simulink model "BLDC_model_My_model"  (R2024b)
settings: Solver=VariableStepAuto  StartTime=0.0  StopTime=2  FixedStep=1e-5  MaxStep=1e-5  RelTol=1e-3
model workspace (MAT data in the model file):
  B = 1e-06
  J = 5e-06
  Ke = 0.0006
  Ls = 2e-05
  Pm = 0.0006
  Rs = 0.06
  f = 50
  p = 8
libraries: spsMosfetLib x6, spsVoltageMeasurementLib x3, dspstat3 x1, slpidlib x1, spsControlledVoltageSourceLib x1, spsDCVoltageSourceLib x1, ee_lib x1, spspowerguiLib x1
settings Model: Creator=ahmed  LastModifiedBy=ahmed

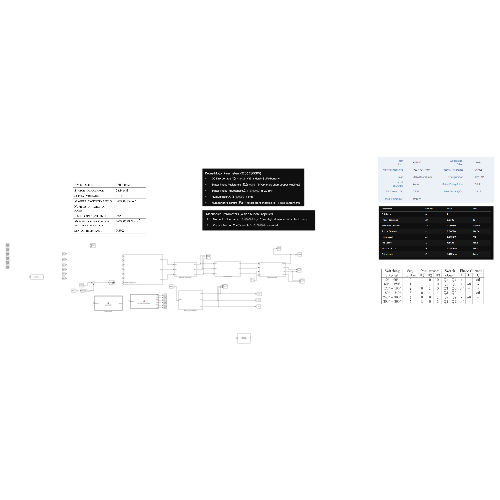
[thumbnail: Simulink's stored preview of the top-level diagram]
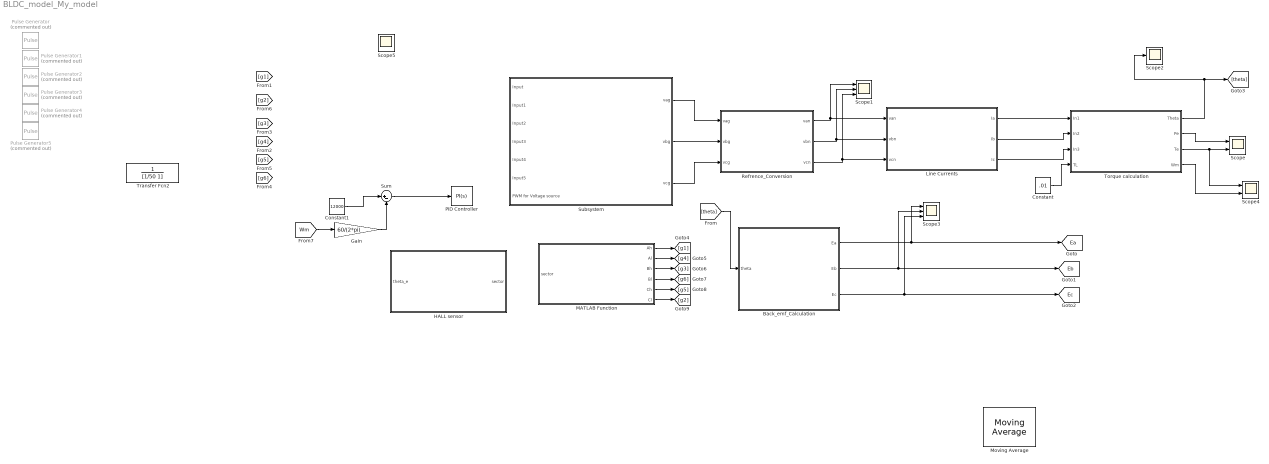
== system BLDC_model_My_model ==
  Back_emf_Calculation : Subsystem
  Constant : Constant  Value=.01
  Constant1 : Constant  Value=12000
  Gain : Gain  Gain=60/(2*pi)
  HALL sensor : MATLAB Function  TreatAsAtomicUnit=on
  Line Currents : Subsystem
  MATLAB Function : MATLAB Function  TreatAsAtomicUnit=on
  Moving Average : dspstat3/Moving Average  Method=Sliding window  ForgettingFactorPort=off  SpecifyWindowLength=on  WindowLength=4  OverlapLength=3  AllowArbitraryInputLength=off  ForgettingFactor=0.9  SimulateUsing=Interpreted execution
  PID Controller : slpidlib/PID Controller  Controller=PI  Form=Parallel  TimeDomain=Continuous-time  UseExternalTs=off  SampleTime=-1  IntegratorMethod=Forward Euler  FilterMethod=Forward Euler  ControllerParametersSource=internal  P=.02  I=600  UseKiTs=off  D=0  UseExternalDerivativeSource=off  N=100  UseFilter=on  TunerSelectOption=Transfer Function Based (PID Tuner App)  InitialConditionSource=internal  InitialConditionForIntegrator=0  InitialConditionForFilter=0  DifferentiatorICPrevScaledInput=0  ExternalReset=none  TrackingMode=off  Kt=1  LimitOutput=on  SatLimitsSource=internal  UpperSaturationLimit=0.636 * 24  LowerSaturationLimit=0  LinearizeAsGain=on  AntiWindupMode=clamping  Kb=1  LimitIntegrator=off  UpperIntegratorSaturationLimit=inf  LowerIntegratorSaturationLimit=-inf  POutMin=[]  POutMax=[]  IOutMin=[]  IOutMax=[]  DOutMin=[]  DOutMax=[]  NOutMin=[]  NOutMax=[]  SumOutMin=[]  SumOutMax=[]  SaturationOutMin=[]  SaturationOutMax=[]  PParamMin=[]  PParamMax=[]  IParamMin=[]  IParamMax=[]  DParamMin=[]  DParamMax=[]  NParamMin=[]  NParamMax=[]  KbParamMin=[]  KbParamMax=[]  KtParamMin=[]  KtParamMax=[]  KbOutMin=[]  KbOutMax=[]  KtOutMin=[]  KtOutMax=[]  IntegratorOutMin=[]  IntegratorOutMax=[]  FilterOutMin=[]  FilterOutMax=[]  SumI1OutMin=[]  SumI1OutMax=[]  SumI2OutMin=[]  SumI2OutMax=[]  SumI3OutMin=[]  SumI3OutMax=[]  SumI4OutMin=[]  SumI4OutMax=[]  SumDOutMin=[]  SumDOutMax=[]  DifferentiatorOutMin=[]  DifferentiatorOutMax=[]  FilterDiffOutCoefMin=[]  FilterDiffOutCoefMax=[]  ReciprocalOutMin=[]  ReciprocalOutMax=[]  SumDenOutMin=[]  SumDenOutMax=[]  SumNumOutMin=[]  SumNumOutMax=[]  DivideOutMin=[]  DivideOutMax=[]  UdiffTsProdOutMin=[]  UdiffTsProdOutMax=[]  NTsProdOutMin=[]  NTsProdOutMax=[]  UintegralTsProdOutMin=[]  UintegralTsProdOutMax=[]  UngainTsProdOutMin=[]  UngainTsProdOutMax=[]  ClampingZeroOutDataTypeStr=Inherit: Inherit via back propagation  ClampingZeroOutMin=[]  ClampingZeroOutMax=[]  FilterDenConstantOutDataTypeStr=Inherit: Inherit via back propagation  FilterDenConstantOutMin=[]  FilterDenConstantOutMax=[]  PCopyOutDataTypeStr=Inherit: Inherit via back propagation  PCopyOutMin=[]  PCopyOutMax=[]  NCopyOutDataTypeStr=Inherit: Inherit via back propagation  NCopyOutMin=[]  NCopyOutMax=[]  IntegratorContinuousStateAttributes=''  IntegratorStateMustResolveToSignalObject=off  IntegratorRTWStateStorageClass=Auto  FilterContinuousStateAttributes=''  FilterStateMustResolveToSignalObject=off  FilterRTWStateStorageClass=Auto  ParallelPVariant=InternalParameters  IdealPVariant=Disabled  IVariant=InternalParameters  DVariant=Disabled  IntegratorVariant=Continuous  SatVariant=Enabled  AWVariant=ContClampingParallel  PCopyVariant=Disabled  TRVariant=Disabled  FdbkBlocksVariant=Forward  IdealPFdbkVariant=Disabled  SatFdbkVariant=Disabled  DerivativeFilterVariant=Disabled  NVariant=Disabled  NCopyVariant=Disabled_SignalSpec  FilterICVariant=Disabled  IntegratorICVariant=InternalICs  ExternalResetVariant=Disabled  TRSumVariant=Passthrough  SumFdbkVariant=Disabled  SumVariant=Sum_PI  TsampFilterVariant=InternalTs  TsampNgainVariant=Passthrough  TsampIntegralVariant=Disabled_SignalSpec  ExternalSaturationOutDataTypeStr=Inherit: Same as second input  DerivativeSourceVariant=Disabled  PreIntVariant=InternalPreInt
  Pulse Generator : DiscretePulseGenerator  Commented=on  PulseType=Time based  Period=1/f  PulseWidth=33
  Pulse Generator1 : DiscretePulseGenerator  Commented=on  PulseType=Time based  Period=1/f  PulseWidth=33  PhaseDelay=2*(1/f)/3
  Pulse Generator2 : DiscretePulseGenerator  Commented=on  PulseType=Time based  Period=1/f  PulseWidth=33  PhaseDelay=(1/f)/3
  Pulse Generator3 : DiscretePulseGenerator  Commented=on  PulseType=Time based  Period=1/f  PulseWidth=33  PhaseDelay=(1/f)/2
  Pulse Generator4 : DiscretePulseGenerator  Commented=on  PulseType=Time based  Period=1/f  PulseWidth=33  PhaseDelay=(1/f)/6
  Pulse Generator5 : DiscretePulseGenerator  Commented=on  PulseType=Time based  Period=1/f  PulseWidth=33  PhaseDelay=5*(1/f)/6
  Refrence_Conversion : Subsystem
  Scope : Scope  NumInputPorts=2
  Scope1 : Scope  NumInputPorts=3
  Scope2 : Scope
  Scope3 : Scope  NumInputPorts=3
  Scope4 : Scope  NumInputPorts=2
  Scope5 : Scope  NumInputPorts=3
  Subsystem : Subsystem
  Sum : Sum  Inputs=|+-
  Torque calculation : Subsystem
  Transfer Fcn2 : TransferFcn  Denominator=[1/50 1]
  tag scope: Ea=global, Eb=global, Ec=global
  wires:
  Subsystem/2(vbg) -> Refrence_Conversion/2(vbg)
  Subsystem/1(vag) -> Refrence_Conversion/1(vag)
  Subsystem/3(vcg) -> Refrence_Conversion/3(vcg)
  Refrence_Conversion/1(van) -> Scope1/1, Line Currents/1(van)
  Refrence_Conversion/2(vbn) -> Scope1/2, Line Currents/2(vbn)
  Refrence_Conversion/3(vcn) -> Scope1/3, Line Currents/3(vcn)
  Line Currents/1(Ia) -> Torque calculation/1(In1)
  Line Currents/2(Ib) -> Torque calculation/2(In2)
  Line Currents/3(Ic) -> Torque calculation/3(In3)
  Torque calculation/1(Theta) -> Scope2/1, [theta]
  Back_emf_Calculation/1(Ea) -> [Ea], Scope3/1
  Back_emf_Calculation/3(Ec) -> [Ec], Scope3/3
  Back_emf_Calculation/2(Eb) -> [Eb], Scope3/2
  MATLAB Function/1(Ah) -> [g1]
  MATLAB Function/2(Al) -> [g4]
  MATLAB Function/3(Bh) -> [g3]
  MATLAB Function/4(Bl) -> [g6]
  MATLAB Function/5(Ch) -> [g5]
  MATLAB Function/6(Cl) -> [g2]
  Torque calculation/2(Pe) -> Scope/1
  Torque calculation/3(Te) -> Scope4/1, Scope/2
  Torque calculation/4(Wm) -> Scope4/2
  Constant/1 -> Torque calculation/4(TL)
  Sum/1 -> PID Controller/1
  [Wm] -> Gain/1
  Gain/1 -> Sum/2
  Constant1/1 -> Sum/1
  [theta] -> Back_emf_Calculation/1(theta)

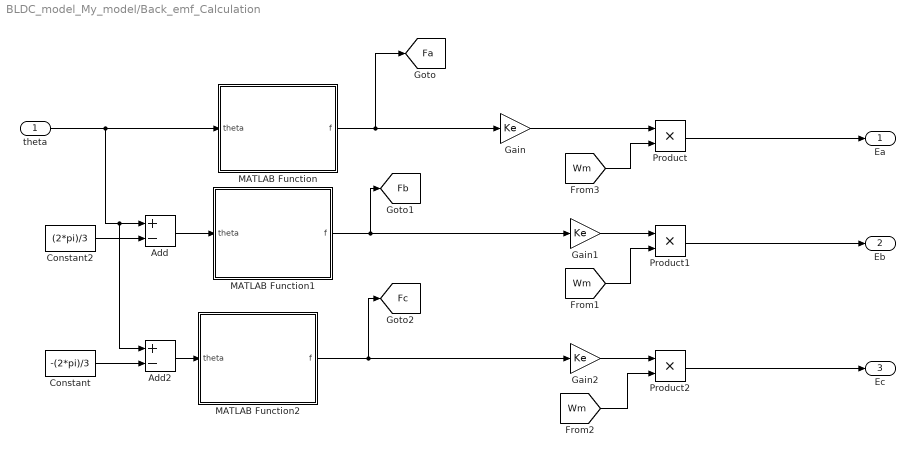
== system BLDC_model_My_model/Back_emf_Calculation ==
  theta : Inport
  Add : Sum  Inputs=+-
  Add2 : Sum  Inputs=+-
  Constant : Constant  Value=-(2*pi)/3
  Constant2 : Constant  Value=(2*pi)/3
  Gain : Gain  Gain=Ke
  Gain1 : Gain  Gain=Ke
  Gain2 : Gain  Gain=Ke
  MATLAB Function : MATLAB Function  TreatAsAtomicUnit=on
  MATLAB Function1 : MATLAB Function  TreatAsAtomicUnit=on
  MATLAB Function2 : MATLAB Function  TreatAsAtomicUnit=on
  Product : Product
  Product1 : Product
  Product2 : Product
  Ea : Outport
  Eb : Outport  Port=2
  Ec : Outport  Port=3
  tag scope: Fa=global, Fb=global, Fc=global
  wires:
  theta/1 -> Add2/1, Add/1, MATLAB Function/1(theta)
  Constant/1 -> Add2/2
  Constant2/1 -> Add/2
  Add/1 -> MATLAB Function1/1(theta)
  Add2/1 -> MATLAB Function2/1(theta)
  MATLAB Function/1(f) -> [Fa], Gain/1
  MATLAB Function1/1(f) -> [Fb], Gain1/1
  MATLAB Function2/1(f) -> [Fc], Gain2/1
  [Wm] -> Product/2
  Gain/1 -> Product/1
  Gain1/1 -> Product1/1
  [Wm] -> Product1/2
  Gain2/1 -> Product2/1
  [Wm] -> Product2/2
  Product/1 -> Ea/1
  Product1/1 -> Eb/1
  Product2/1 -> Ec/1

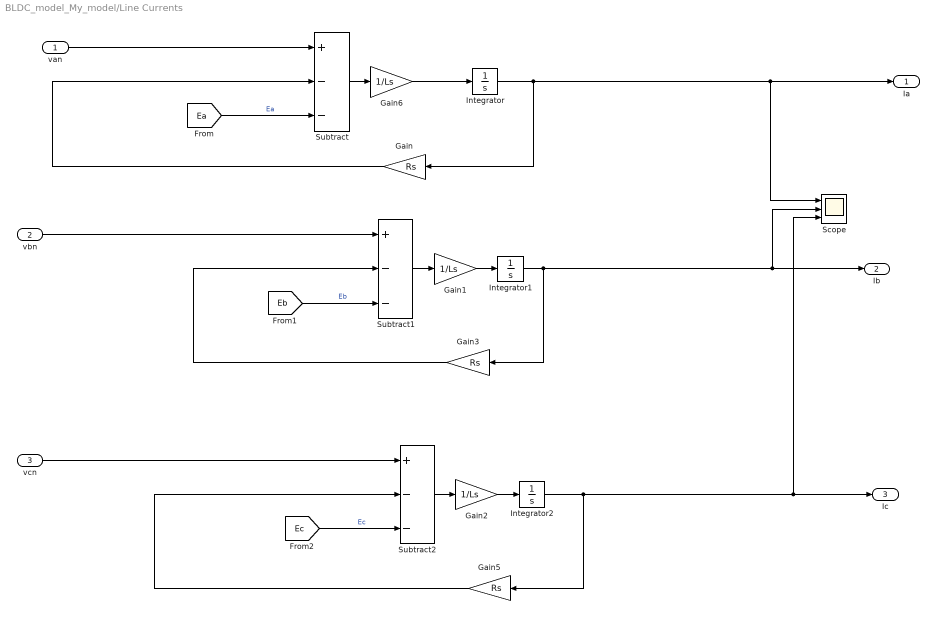
== system BLDC_model_My_model/Line Currents ==
  van : Inport
  vbn : Inport  Port=2
  vcn : Inport  Port=3
  Gain : Gain  Gain=Rs
  Gain1 : Gain  Gain=1/Ls
  Gain2 : Gain  Gain=1/Ls
  Gain3 : Gain  Gain=Rs
  Gain5 : Gain  Gain=Rs
  Gain6 : Gain  Gain=1/Ls
  Integrator : Integrator
  Integrator1 : Integrator
  Integrator2 : Integrator
  Scope : Scope  NumInputPorts=3
  Subtract : Sum  Inputs=+--
  Subtract1 : Sum  Inputs=+--
  Subtract2 : Sum  Inputs=+--
  Ia : Outport
  Ib : Outport  Port=2
  Ic : Outport  Port=3
  wires:
  van/1 -> Subtract/1
  [Ea] -> Subtract/3  "Ea"
  Subtract/1 -> Gain6/1
  Gain/1 -> Subtract/2
  Integrator/1 -> Scope/1, Ia/1, Gain/1
  Gain3/1 -> Subtract1/2
  Subtract1/1 -> Gain1/1
  vbn/1 -> Subtract1/1
  vcn/1 -> Subtract2/1
  Subtract2/1 -> Gain2/1
  Gain5/1 -> Subtract2/2
  [Eb] -> Subtract1/3  "Eb"
  [Ec] -> Subtract2/3  "Ec"
  Integrator2/1 -> Ic/1, Scope/3, Gain5/1
  Integrator1/1 -> Scope/2, Ib/1, Gain3/1
  Gain6/1 -> Integrator/1
  Gain1/1 -> Integrator1/1
  Gain2/1 -> Integrator2/1

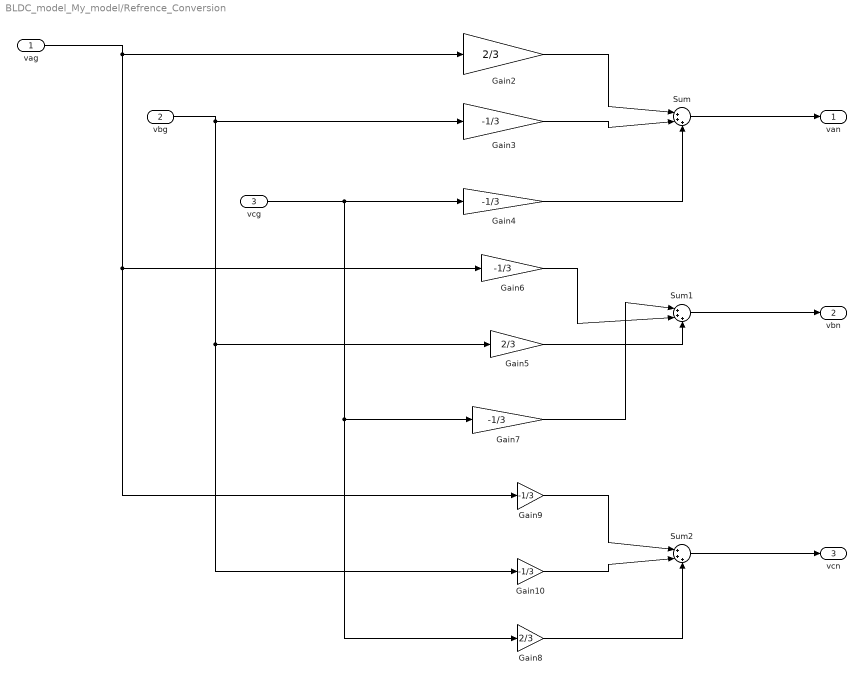
== system BLDC_model_My_model/Refrence_Conversion ==
  vag : Inport
  vbg : Inport  Port=2
  vcg : Inport  Port=3
  Gain{3..4,6..7,9..10} (6 alike) : Gain  Gain=-1/3
  Gain2 : Gain  Gain=2/3
  Gain5 : Gain  Gain=2/3
  Gain8 : Gain  Gain=2/3
  Sum : Sum  Inputs=|+++
  Sum1 : Sum  Inputs=|+++
  Sum2 : Sum  Inputs=|+++
  van : Outport
  vbn : Outport  Port=2
  vcn : Outport  Port=3
  wires:
  Gain10/1 -> Sum2/2
  Gain9/1 -> Sum2/1
  Gain8/1 -> Sum2/3
  Gain7/1 -> Sum1/1
  Gain4/1 -> Sum/3
  Gain3/1 -> Sum/2
  vbg/1 -> Gain10/1, Gain5/1, Gain3/1
  Gain6/1 -> Sum1/2
  Gain2/1 -> Sum/1
  vcg/1 -> Gain8/1, Gain7/1, Gain4/1
  Gain5/1 -> Sum1/3
  vag/1 -> Gain2/1, Gain6/1, Gain9/1
  Sum/1 -> van/1
  Sum1/1 -> vbn/1
  Sum2/1 -> vcn/1

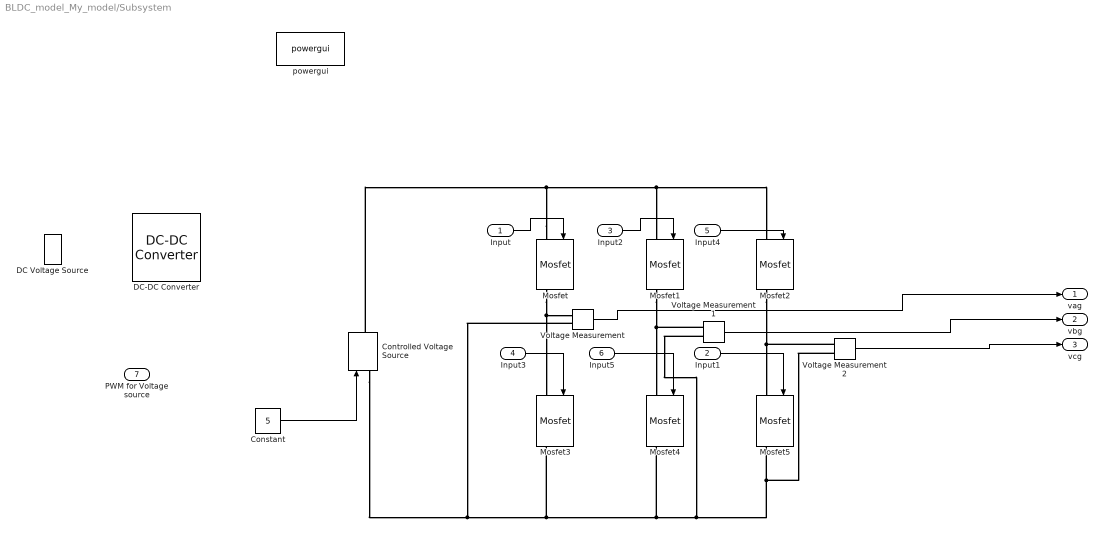
== system BLDC_model_My_model/Subsystem ==
  Input : Inport
  Input1 : Inport  Port=2
  Input2 : Inport  Port=3
  Input3 : Inport  Port=4
  Input4 : Inport  Port=5
  Input5 : Inport  Port=6
  PWM for Voltage source : Inport  Port=7
  Constant : Constant  Value=5
  Controlled Voltage Source : spsControlledVoltageSourceLib/Controlled Voltage Source  Initialize=on  Source_Type=DC  Amplitude=0  Phase=0  Frequency=0  Measurements=Voltage
  DC Voltage Source : spsDCVoltageSourceLib/DC Voltage Source  Amplitude=100  Measurements=None
  DC-DC Converter : ee_lib/Semiconductors & Converters/Converters/DC-DC Converter  Vref_option=ee.enum.converters.voltageref.internal  v_ref=10 V  P_rated=10 W  droop_enabled=true  droop_param=ee.enum.converters.droop.value  droop=0.1 V/A  droop_percent=2  Vref_droop=10 V  reversible=ee.enum.converters.directionality.unidirectional  G_diode=1e-8 1/Ohm  P_fixed=1 W  losses_option=ee.enum.converters.lossesOption.proportionalToSquaredCurrent  eff_rated=80  tableOption=ee.enum.converters.lossTableOptionThermal.currentTemp  i_eff_vec=[-2, -1, 1, 2] A  v_eff_vec=[15, 30, 45] V  eff_vec=[66, 76, 80, 74]  eff_2D_table=[66, 66, 66; 76, 76, 76; 80, 80, 80; 74, 74, 74]  model_dynamics=ee.enum.converters.dynamics.no  tau=0.02 s  v_ini=10 V  v1_min=1 V  R1=1000 Ohm  R2=1000 Ohm  fault_condition=ee.enum.faults.faultInputCondition.greaterThan  fault_threshold=0.5  T_eff_vec=[280, 300, 320] K  eff_3D_table=repmat([66; 76; 80; 74], 1, 3, 3)  thermal_mass=100 J/K  initial_temperature=298.15 K
      settings: InternalSimscapePortConfiguration="{\"Bottom\":[],\"Left\":[{\"id\":\"p1\",\"label\":\"1+\",\"type\":\"foundation.electrical.electrical\"},{\"id\":\"n1\",\"label\":\"1-\",\"type\":\"foundation.electrical.electrical\"}],\"Right\":[{\"id\":\"p2\",\"label\":\"2+\",\"type\":\"foundation.electrical.electrical\"},{\"id\":\"n2\",\"label\":\"2-\",\"type\":\"foundation.electrical.electrical\"}],\"Top\":[]}"
  Mosfet{,1..5} (6 alike) : spsMosfetLib/Mosfet  Ron=0.1  Lon=0  Rd=0.01  Vfd=0  IC=0  Rs=1e5  Cs=inf  Measurements=on
  Voltage Measurement : spsVoltageMeasurementLib/Voltage Measurement  PhasorSimulation=off  OutputType=Complex  PSBequivalent=0
  Voltage Measurement1 : spsVoltageMeasurementLib/Voltage Measurement  PhasorSimulation=off  OutputType=Complex  PSBequivalent=0
  Voltage Measurement2 : spsVoltageMeasurementLib/Voltage Measurement  PhasorSimulation=off  OutputType=Complex  PSBequivalent=0
  powergui : spspowerguiLib/powergui  Priority=1  SimulationMode=Continuous  SampleTime=50e-6  frequency=60  Iterations=50  frequencyindice=0  Pbase=100e6  ErrMax=1e-4  UnitsV=kV  UnitsW=MW  buscounter=0  FunctionMessages=off  echomessages=off  EnableUseOfTLC=off  CurrentSourceSwitches=off  DisableSnubberDevices=off  DisableRonSwitches=off  DisableVfSwitches=off  DisplayEquations=off  AutomaticDiscreteSolvers=off  SolverType=Tustin/Backward Euler (TBE)  Interpol=off  ExternalGateDelay=off  methode=off  Ts=100  x0status=blocks  SPID=on  SwTol=0  HookPort=off  NonlinearTolerance=1e-4  nMaxIteration=100  ContinueOnMaxIteration=off  RestoreLinks=warning  ResistiveCurrentMeasurement=off  Frange=[0:2:500]  Ylog=off  Xlog=on  ShowGrid=off  save=off  variable=ZData  structure=0  ZoomFFT=off  StartTime=0.0  cycles=1  DisplayStyle=1  fundamental=60  FreqAxis=off  MaxFrequency=1000  frequencyindicesteady=1  RmsSteady=1  display=off
  vag : Outport
  vbg : Outport  Port=2
  vcg : Outport  Port=3
  wires:
  Input2/1 -> Mosfet1/1
  Input5/1 -> Mosfet4/1
  Voltage Measurement1/1 -> vbg/1
  Input4/1 -> Mosfet2/1
  Input/1 -> Mosfet/1
  Voltage Measurement/1 -> vag/1
  Input3/1 -> Mosfet3/1
  Input1/1 -> Mosfet5/1
  Voltage Measurement2/1 -> vcg/1
  Constant/1 -> Controlled Voltage Source/1
  connections:
  Mosfet/LConn1 -- Controlled Voltage Source/RConn1 -- Mosfet1/LConn1 -- Mosfet2/LConn1
  Controlled Voltage Source/LConn1 -- Voltage Measurement/LConn2 -- Mosfet3/RConn1 -- Voltage Measurement1/LConn2 -- Voltage Measurement2/LConn2 -- Mosfet5/RConn1 -- Mosfet4/RConn1
  Mosfet2/RConn1 -- Voltage Measurement2/LConn1 -- Mosfet5/LConn1
  Mosfet1/RConn1 -- Voltage Measurement1/LConn1 -- Mosfet4/LConn1
  Mosfet/RConn1 -- Mosfet3/LConn1 -- Voltage Measurement/LConn1

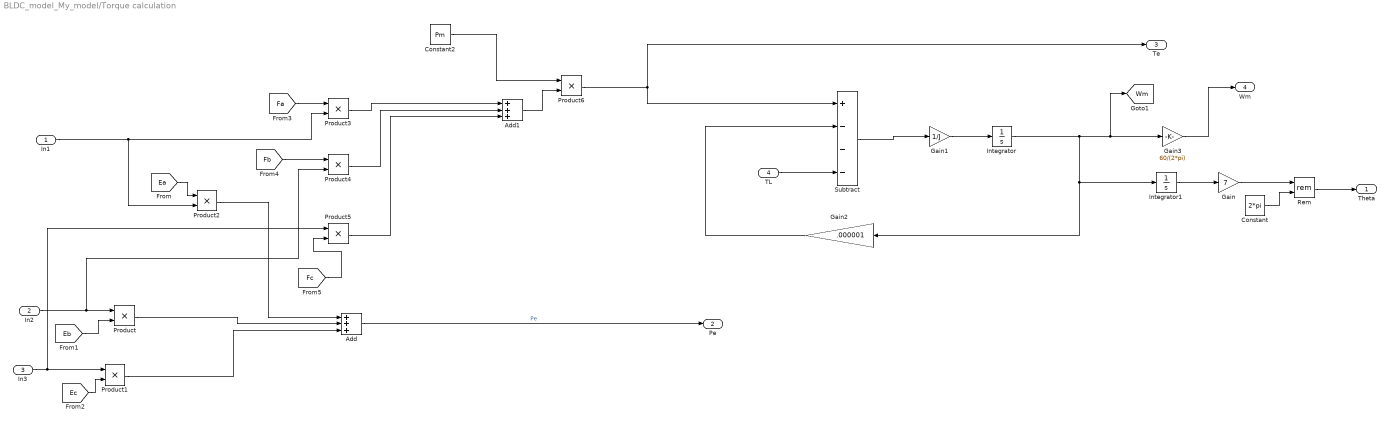
== system BLDC_model_My_model/Torque calculation ==
  In1 : Inport
  In2 : Inport  Port=2
  In3 : Inport  Port=3
  TL : Inport  Port=4
  Add : Sum  Inputs=+++
  Add1 : Sum  Inputs=+++
  Constant : Constant  Value=2*pi
  Constant2 : Constant  Value=Pm
  Gain : Gain  Gain=7
  Gain1 : Gain  Gain=1/J
  Gain2 : Gain  Gain=.000001
  Gain3 : Gain  Gain=60/(2*pi)
  Integrator : Integrator
  Integrator1 : Integrator
  Product{,1..6} (7 alike) : Product
  Rem : Math  Operator=rem
  Subtract : Sum  Inputs=+---
  Theta : Outport
  Pe : Outport  Port=2
  Te : Outport  Port=3
  Wm : Outport  Port=4
  tag scope: Wm=global
  wires:
  In2/1 -> Product4/2, Product/1
  [Eb] -> Product/2
  In3/1 -> Product1/1, Product5/1
  [Ec] -> Product1/2
  [Ea] -> Product2/1
  In1/1 -> Product2/2, Product3/2
  Product2/1 -> Add/1
  Product/1 -> Add/2
  Product1/1 -> Add/3
  Add/1 -> Pe/1  "Pe"
  Integrator1/1 -> Gain/1
  Gain/1 -> Rem/1
  Constant/1 -> Rem/2
  Rem/1 -> Theta/1
  Subtract/1 -> Gain1/1
  Gain1/1 -> Integrator/1
  Integrator/1 -> [Wm], Gain3/1, Integrator1/1, Gain2/1
  Gain2/1 -> Subtract/2
  TL/1 -> Subtract/4
  [Fa] -> Product3/1
  [Fb] -> Product4/1
  [Fc] -> Product5/2
  Product3/1 -> Add1/1
  Product4/1 -> Add1/2
  Product5/1 -> Add1/3
  Add1/1 -> Product6/2
  Constant2/1 -> Product6/1
  Product6/1 -> Te/1, Subtract/1
  Gain3/1 -> Wm/1

== matlab function BLDC_model_My_model/Back_emf_Calculation/MATLAB Function1 ==
  data: theta input; f output
function f = calc_f_standard(theta)
    % calc_f_standard calculates the unit trapezoidal back-EMF waveform 
    % based on the standard literature formulation (starts at the flat top).
    %
    % Input: theta - Electrical angle in radians (can be scalar or array)
    % Output: f - Normalized back-EMF amplitude (-1.0 to 1.0)
    
    % Normalize angle to strictly fall within [0, 2*pi)
    theta_norm = mod(theta, 2*pi);
    
    % Initialize the output array with zeros
    f = zeros(size(theta_norm));
    
    % Region 1: Flat Top (0 to 120 degrees)
    idx = (theta_norm >= 0) & (theta_norm < 2*pi/3);
    f(idx) = 1;
    
    % Region 2: Falling Edge (120 to 180 degrees)
    idx = (theta_norm >= 2*pi/3) & (theta_norm < pi);
    f(idx) = 1 - (6/pi) .* (theta_norm(idx) - 2*pi/3);
    
    % Region 3: Flat Bottom (180 to 300 degrees)
    idx = (theta_norm >= pi) & (theta_norm < 5*pi/3);
    f(idx) = -1;
    
    % Region 4: Rising Edge (300 to 360 degrees)
    idx = (theta_norm >= 5*pi/3) & (theta_norm <= 2*pi);
    f(idx) = -1 + (6/pi) .* (theta_norm(idx) - 5*pi/3);
end

== matlab function BLDC_model_My_model/Back_emf_Calculation/MATLAB Function ==
  data: theta input; f output
function f = calc_f_standard(theta)
    % calc_f_standard calculates the unit trapezoidal back-EMF waveform 
    % based on the standard literature formulation (starts at the flat top).
    %
    % Input: theta - Electrical angle in radians (can be scalar or array)
    % Output: f - Normalized back-EMF amplitude (-1.0 to 1.0)
    
    % Normalize angle to strictly fall within [0, 2*pi)
    theta_norm = mod(theta, 2*pi);
    
    % Initialize the output array with zeros
    f = zeros(size(theta_norm));
    
    % Region 1: Flat Top (0 to 120 degrees)
    idx = (theta_norm >= 0) & (theta_norm < 2*pi/3);
    f(idx) = 1;
    
    % Region 2: Falling Edge (120 to 180 degrees)
    idx = (theta_norm >= 2*pi/3) & (theta_norm < pi);
    f(idx) = 1 - (6/pi) .* (theta_norm(idx) - 2*pi/3);
    
    % Region 3: Flat Bottom (180 to 300 degrees)
    idx = (theta_norm >= pi) & (theta_norm < 5*pi/3);
    f(idx) = -1;
    
    % Region 4: Rising Edge (300 to 360 degrees)
    idx = (theta_norm >= 5*pi/3) & (theta_norm <= 2*pi);
    f(idx) = -1 + (6/pi) .* (theta_norm(idx) - 5*pi/3);
end

== matlab function BLDC_model_My_model/Back_emf_Calculation/MATLAB Function2 ==
  data: theta input; f output
function f = calc_f_standard(theta)
    % calc_f_standard calculates the unit trapezoidal back-EMF waveform 
    % based on the standard literature formulation (starts at the flat top).
    %
    % Input: theta - Electrical angle in radians (can be scalar or array)
    % Output: f - Normalized back-EMF amplitude (-1.0 to 1.0)
    
    % Normalize angle to strictly fall within [0, 2*pi)
    theta_norm = mod(theta, 2*pi);
    
    % Initialize the output array with zeros
    f = zeros(size(theta_norm));
    
    % Region 1: Flat Top (0 to 120 degrees)
    idx = (theta_norm >= 0) & (theta_norm < 2*pi/3);
    f(idx) = 1;
    
    % Region 2: Falling Edge (120 to 180 degrees)
    idx = (theta_norm >= 2*pi/3) & (theta_norm < pi);
    f(idx) = 1 - (6/pi) .* (theta_norm(idx) - 2*pi/3);
    
    % Region 3: Flat Bottom (180 to 300 degrees)
    idx = (theta_norm >= pi) & (theta_norm < 5*pi/3);
    f(idx) = -1;
    
    % Region 4: Rising Edge (300 to 360 degrees)
    idx = (theta_norm >= 5*pi/3) & (theta_norm <= 2*pi);
    f(idx) = -1 + (6/pi) .* (theta_norm(idx) - 5*pi/3);
end

== matlab function BLDC_model_My_model/MATLAB Function ==
  data: sector input; Ah output; Al output; Bh output; Bl output; Ch output; Cl output
function [Ah, Al, Bh, Bl, Ch, Cl] = six_step_commutation(sector)
    % six_step_commutation maps the active 60-degree sector directly to the 
    % 3-phase inverter gate signals for pure 120-degree block commutation.
    % (No PWM chopping applied, purely solid ON/OFF states).
    %
    % Inputs: 
    %   sector - The active commutation sector (1 through 6)
    %            Can be a scalar or an array of values.
    %
    % Outputs: 
    %   Ah, Bh, Ch - Upper gate signals for Phases A, B, C (1 = ON, 0 = OFF)
    %   Al, Bl, Cl - Lower gate signals for Phases A, B, C (1 = ON, 0 = OFF)
    
    % 1. Initialize all gates to OFF (0) to prevent shoot-through
    Ah = zeros(size(sector)); Al = zeros(size(sector));
    Bh = zeros(size(sector)); Bl = zeros(size(sector));
    Ch = zeros(size(sector)); Cl = zeros(size(sector));
    
    % 2. Vectorized Switch-Case logic for all 6 sectors
    % Sector 1: Phase A Active (+), Phase B Return (-)
    idx = (sector == 1);
    if any(idx)
        Ah(idx) = 1; 
        Bl(idx) = 1; 
    end
    
    % Sector 2: Phase A Active (+), Phase C Return (-)
    idx = (sector == 2);
    if any(idx)
        Ah(idx) = 1; 
        Cl(idx) = 1; 
    end
    
    % Sector 3: Phase B Active (+), Phase C Return (-)
    idx = (sector == 3);
    if any(idx)
        Bh(idx) = 1; 
        Cl(idx) = 1; 
    end
    
    % Sector 4: Phase B Active (+), Phase A Return (-)
    idx = (sector == 4);
    if any(idx)
        Bh(idx) = 1; 
        Al(idx) = 1; 
    end
    
    % Sector 5: Phase C Active (+), Phase A Return (-)
    idx = (sector == 5);
    if any(idx)
        Ch(idx) = 1; 
        Al(idx) = 1; 
    end
    
    % Sector 6: Phase C Active (+), Phase B Return (-)
    idx = (sector == 6);
    if any(idx)
        Ch(idx) = 1; 
        Bl(idx) = 1; 
    end
end

== matlab function BLDC_model_My_model/HALL sensor ==
  data: theta_e input; sector output
function sector = get_sector(theta_e)
    % Directly calculates the commutation sector (1-6) from the electrical angle.
    % Bypasses the need for physical Hall Effect sensor logic in pure simulations.
    
    % 1. Normalize angle to strictly fall within [0, 2*pi)
    theta_norm = mod(theta_e, 2*pi);
    
    % =========================================================================
    % THE SIX CASES (Mathematical Domains)
    % =========================================================================
    % Case 1: 0° to 60°     (0 to pi/3 rad)       --> Sector = 1
    % Case 2: 60° to 120°   (pi/3 to 2*pi/3 rad)  --> Sector = 2
    % Case 3: 120° to 180°  (2*pi/3 to pi rad)    --> Sector = 3
    % Case 4: 180° to 240°  (pi to 4*pi/3 rad)    --> Sector = 4
    % Case 5: 240° to 300°  (4*pi/3 to 5*pi/3 rad)--> Sector = 5
    % Case 6: 300° to 360°  (5*pi/3 to 2*pi rad)  --> Sector = 6
    
    % =========================================================================
    % 2. Calculate the Sector
    % Instead of writing 6 if/else statements, this single line of math 
    % safely categorizes any angle into the correct 1 through 6 sector.
    % =========================================================================
    sector = floor(theta_norm / (pi/3)) + 1;
    
end
